simulink subsystem "Inputs_BatteryHV_refsub"  (R2026a)
settings: Solver=VariableStepAuto
PreLoadFcn:
  | batteryHV.Input_LoadCurrent_Data = simscape.Value([0 0 0], "A");
  | batteryHV.Input_LoadCurrent_TimePoints = simscape.Value([0 1 2], "s");
  | 
  | batteryHV.Input_HeatFlow_Data = simscape.Value([0 0 0], "W");
  | batteryHV.Input_HeatFlow_TimePoints = simscape.Value([0 1 2], "s");
libraries: simulink x1
settings Model: Creator=isaacito  LastModifiedBy=isaacito
settings SimscapeCC: SimscapeNominalValues="[{\"value\":\"1\",\"unit\":\"A\"},{\"value\":\"1\",\"unit\":\"bar\"},{\"value\":\"1\",\"unit\":\"cm^2\"},{\"value\":\"1\",\"unit\":\"cm^3/s\"},{\"value\":\"1\",\"unit\":\"kJ/kg\"},{\"value\":\"1\",\"unit\":\"kW\"},{\"value\":\"1\",\"unit\":\"l\"},{\"value\":\"1\",\"unit\":\"N\"},{\"value\":\"1\",\"unit\":\"N*m\"},{\"value\":\"1\",\"unit\":\"V\"}]"  SimscapeLogType=none  SimscapeLogDataHistory=5000.0

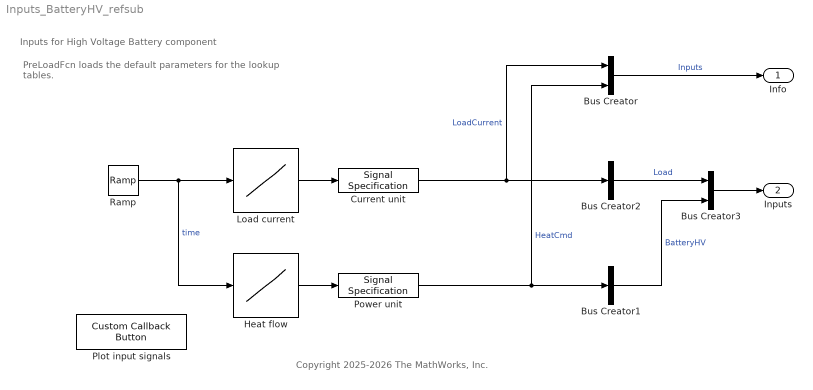
== system Inputs_BatteryHV_refsub ==
  note: PreLoadFcn loads the default parameters
      | for the lookup tables.
  note: Copyright 2025-2026 The MathWorks, Inc.
  note: Inputs for High Voltage Battery component
  Bus Creator : BusCreator  Inputs=2
  Bus Creator1 : BusCreator  Inputs=1
  Bus Creator2 : BusCreator  Inputs=1
  Bus Creator3 : BusCreator  Inputs=2
  Current unit : SignalSpecification  Unit=A
  Heat flow : Lookup_n-D  NumberOfTableDimensions=1  BreakpointsForDimension1="batteryHV.Input_HeatFlow_TimePoints.value(\"s\")"  Table="batteryHV.Input_HeatFlow_Data.value(\"W\")"  InterpMethod=Akima spline  InternalRulePriority=Speed  RndMeth=Simplest
  Load current : Lookup_n-D  NumberOfTableDimensions=1  BreakpointsForDimension1="batteryHV.Input_LoadCurrent_TimePoints.value(\"s\")"  Table="batteryHV.Input_LoadCurrent_Data.value(\"A\")"  InterpMethod=Akima spline  InternalRulePriority=Speed  RndMeth=Simplest
  Plot input signals : CustomCallbackButton  Configuration="{\"components\":[{\"name\":\"BackgroundImageComponent\",\"settings\":{\"image\":{\"size\":[0,0],\"src\":\"default\",\"srcOrientation\":\"Right\"},\"position\":[0,0,1,1]}},{\"name\":\"ButtonStateComponent\",\"settings\":{\"buttonType\":\"momentary\",\"clickFcn\":\"bevutil1.SignalUtil.plotLookupTable1DBlocks(gcs, Blocks=[\\\"\\/Load current\\\"; \\\"\\/Heat flow\\\"], DivisionType=\\\"InterpolationInterval\\\", InterpolationInterval=0.2)\",\"onValue\":1,\"position\":[0,0,1,1],\"pressDelay\":\"500\",\"pressFcn\":\"\",\"repeatInterval\":\"0\",\"states\":[{\"horizontalAlignment\":\"center\",\"image\":{\"position\":[0,0,1,1],\"size\":[1,1],\"src\":\"default\",\"srcOrientation\":\"Right\"},\"label\":{\"color\":[0.01176470588,0.01176470588,0.01176470588,1],\"icon\":{\"size\":[0,0],\"src\":\"default\",\"srcOrientation\":\"Right\"},\"iconOffset\":0,\"iconPlacement\":\"left\",\"opacity\":1,\"show\":true,\"text\":{\"content\":\"Plot LUTs\",\"font\":\"Helvetica\"}},\"labelOffset\":[0,0],\"verticalAlignment\":\"middle\"},{\"horizontalAlignment\":\"center\",\"image\":{\"position\":[0,0,1,1],\"size\":[1,1],\"src\":\"default\",\"srcOrientation\":\"Right\"},\"label\":{\"color\":[0.01176470588,0.01176470588,0.01176470588,1],\"icon\":{\"size\":[0,0],\"src\":\"default\",\"srcOrientation\":\"Right\"},\"iconOffset\":0,\"iconPlacement\":\"left\",\"opacity\":1,\"show\":true,\"text\":{\"content\":\"Plot LUTs\",\"font\":\"Helvetica\"}},\"labelOffset\":[0,0],\"verticalAlignment\":\"middle\"},{\"horizontalAlignment\":\"center\",\"image\":{\"position\":[0,0,1,1],\"size\":[1,1],\"src\":\"default\",\"srcOrientation\":\"Right\"},\"label\":{\"color\":[0.01176470588,0.01176470588,0.01176470588,1],\"icon\":{\"size\":[0,0],\"src\":\"default\",\"srcOrientation\":\"Right\"},\"iconOffset\":0,\"iconPlacement\":\"left\",\"opacity\":1,\"show\":true,\"text\":{\"content\":\"Plot LUTs\",\"font\":\"Helvetica\"}},\"labelOffset\":[0,0],\"verticalAlignment\":\"middle\"},{\"horizontalAlignment\":\"center\",\"image\":{\"position\":[0,0,1,1],\"size\":[1,1],\"src\":\"default\",\"srcOrientation\":\"Right\"},\"label\":{\"color\":[0.01176470588,0.01176470588,0.01176470588,1],\"icon\":{\"size\":[0,0],\"src\":\"default\",\"srcOrientation\":\"Right\"},\"iconOffset\":0,\"iconPlacement\":\"left\",\"opacity\":1,\"show\":true,\"text\":{\"content\":\"Plot LUTs\",\"font\":\"Helvetica\"}},\"labelOffset\":[0,0],\"verticalAlignment\":\"middle\"}]}},{\"name\":\"ForegroundImageComponent\",\"settings\":{\"image\":{\"size\":[0,0],\"src\":\"default\",\"srcOrientation\":\"Right\"},\"isForeground\":1,\"position\":[0,0,1,1]}}],\"derived\":{\"blockParameters\":{\"AutoActivate\":true,\"ButtonText\":\"Plot LUTs\",\"ButtonType\":\"Momentary\",\"ClickFcn\":\"bevutil1.SignalUtil.plotLookupTable1DBlocks(gcs, Blocks=[\\\"\\/Load current\\\"; \\\"\\/Heat flow\\\"], DivisionType=\\\"InterpolationInterval\\\", InterpolationInterval=0.2)\",\"OnValue\":1,\"PressDelay\":\"500\",\"PressFcn\":\"\",\"RepeatInterval\":\"0\",\"fixedAspectRatio\":\"off\"}},\"settings\":{\"BindingType\":\"standalone\",\"autoActivate\":true,\"backgroundColor\":[244,244,244,1],\"backgroundOffset\":0.2,\"backgroundOpacity\":1,\"fixedAspectRatio\":\"off\",\"foregroundColor\":[0.01176470588,0.01176470588,0.01176470588,1],\"migratedFromLegacy\":true,\"useBackgroundColor\":true,\"variant\":\"callback\",\"version\":\"R2025a\"},\"type\":\"Button\"}"  CustomBackgroundColor="{\"color\":[0.9568627451,0.9568627451,0.9568627451],\"show\":true}"
  Power unit : SignalSpecification  Unit=W
  Ramp : simulink/Sources/Ramp  slope=1  start=0  InitialOutput=0
      settings: AttributesFormatString=|
      | Slope: %<slope>
      | Start time: %<start>
      | Initial output: %<InitialOutput>
  Info : Outport
  Inputs : Outport  Port=2
  wires:
  Bus Creator/1 -> Info/1  "Inputs"
  Load current/1 -> Current unit/1
  Bus Creator1/1 -> Bus Creator3/2  "BatteryHV"
  Bus Creator2/1 -> Bus Creator3/1  "Load"
  Bus Creator3/1 -> Inputs/1
  Ramp/1 -> Heat flow/1, Load current/1  "time"
  Current unit/1 -> Bus Creator2/1, Bus Creator/1  "LoadCurrent"
  Heat flow/1 -> Power unit/1
  Power unit/1 -> Bus Creator1/1, Bus Creator/2  "HeatCmd"
